simulink model "UDB4_TestBoard"  (Simulink 7.8)
settings: Solver=FixedStepDiscrete  SolverMode=SingleTasking  StartTime=0.0  StopTime=inf  FixedStep=0.001  RelTol=1e-3
libraries: dsPICdrivers x13, simulink x11
settings Model: Creator=Lior  LastModifiedBy=M91449  BufferReuse=off
settings OptimizationCC: BlockReduction=off  InlineParams=on  BufferReuse=off  OptimizeModelRefInitCode=on  LifeSpan=1
settings DebuggingCC: FcnCallInpInsideContextMsg=Use local settings
settings HardwareCC: ProdBitPerInt=16  ProdBitPerPointer=16  ProdEndianess=LittleEndian  ProdWordSize=16  ProdHWDeviceType=16-bit Generic
settings RTWCC: SystemTargetFile=dspic.tlc  MakeCommand=make_CreateMPLAB  TemplateMakefile=dspic_pic30_gcc.tmf  PostCodeGenCommand=dsPIC_Compile()  Description=Embedded Target for Microchip dsPIC (real-time)  ProcessScript=dspic_make_rtw_hook
settings CodeAppCC: IgnoreCustomStorageClasses=off
settings STFCustomTargetCC: IncludeMdlTerminateFcn=off  GeneratePreprocessorConditionals=Use local settings  CombineOutputUpdateFcns=on  SuppressErrorStatus=on  ERTCustomFileBanners=on  SupportContinuousTime=off  SupportNonInlinedSFcns=off  SystemTargetFile=dspic.tlc
settings ERTTargetCC: MultiwordLength=2048  ParMdlRefBuildCompliant=off  CompOptLevelCompliant=off  ConcurrentExecutionCompliant=off  IncludeMdlTerminateFcn=off  SuppressErrorStatus=on  ERTFirstTimeCompliant=off  ModelStepFunctionPrototypeControlCompliant=off  CPPClassGenCompliant=off  ExtModeMexFile=noextcomm  InlinedParameterPlacement=NonHierarchical  ERTSrcFileBannerTemplate=dsPIC_code_template.cgt  ERTHdrFileBannerTemplate=dsPIC_code_template.cgt  ERTDataSrcFileTemplate=dsPIC_code_template.cgt  ERTDataHdrFileTemplate=dsPIC_code_template.cgt  ERTCustomFileTemplate=dsPIC_main.tlc  ConvertIfToSwitch=off  SuppressUnreachableDefaultCases=off
settings CustomProperty: DataType=string  Value=C:\PROGRA~1\MATLAB\R2011B~1\bin\win64\gmake

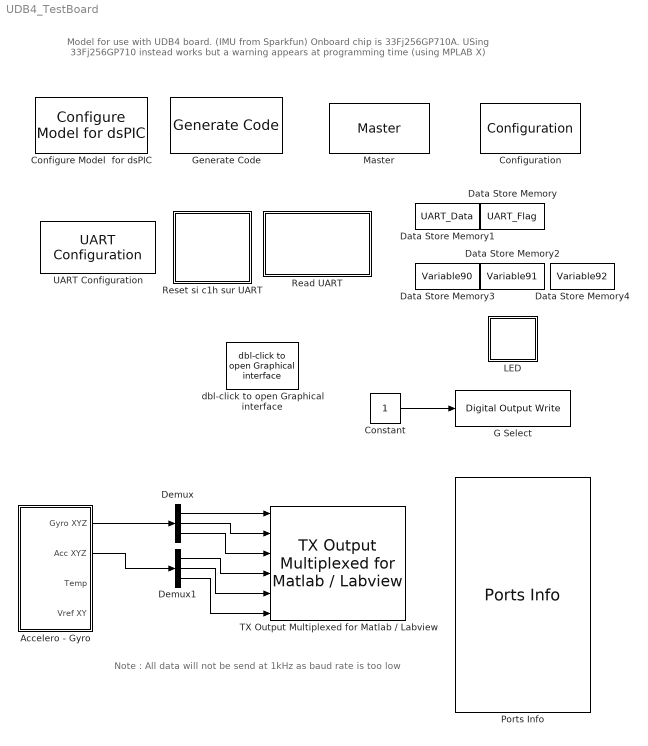
== system UDB4_TestBoard ==
  note: Model for use with UDB4 board. (IMU from Sparkfun)
      | Onboard chip is 33Fj256GP710A.
      | USing 33Fj256GP710 instead works but a warning appears at programming time (using MPLAB X)
  note: Note : All data will not be send at 1kHz as baud rate is too low
  Accelero - Gyro : Subsystem
  Configuration : dsPICdrivers/Configuration  double64=off
  Configure Model  for dsPIC : dsPICdrivers/Simulink Configuration/Configure Model  for dsPIC
  Constant : Constant  OutDataTypeStr=Inherit: Inherit via back propagation
  Data Store Memory : DataStoreMemory  DataStoreName=UART_Flag  ReadBeforeWriteMsg=warning  WriteAfterWriteMsg=warning  WriteAfterReadMsg=warning
  Data Store Memory1 : DataStoreMemory  DataStoreName=UART_Data  ReadBeforeWriteMsg=warning  WriteAfterWriteMsg=warning  WriteAfterReadMsg=warning
  Data Store Memory2 : DataStoreMemory  DataStoreName=Variable91  ReadBeforeWriteMsg=warning  WriteAfterWriteMsg=warning  WriteAfterReadMsg=warning  OutDataTypeStr=uint8
  Data Store Memory3 : DataStoreMemory  DataStoreName=Variable90  ReadBeforeWriteMsg=warning  WriteAfterWriteMsg=warning  WriteAfterReadMsg=warning  OutDataTypeStr=uint8
  Data Store Memory4 : DataStoreMemory  DataStoreName=Variable92  ReadBeforeWriteMsg=warning  WriteAfterWriteMsg=warning  WriteAfterReadMsg=warning  OutDataTypeStr=uint8
  Demux : Demux  Outputs=3
  Demux1 : Demux  Outputs=3
  G Select : dsPICdrivers/Digital I//O/Digital Output Write  Tag=dsPIC_Digital_Output  Priority=5  PORT=A  Pin=6  Simultaneous=on  OrderingInOutPopup=None
  Generate Code : dsPICdrivers/Simulink Configuration/Generate Code
  LED : Subsystem
  Master : dsPICdrivers/Master  Tag=dsPIC_MASTER  Priority=1  TimeStepType=Timer1  picType=33fJ256GP710  fcy=22111111.1111  Quartz_33f=8e6  PLLActive_33f=on  fcyDesired_33f=7.37e6*3  tmr1="[1  22110  0.00050251]"  tmr1Info="Time Step : 0.00099999  ;   Error : 0.00050251%  PR1=22110"  tmr2345="[0  0  0  0  0  0  0  0]"  tmr2345cfg=[-1 -1 -1 -1 -1 -1 -1 -1]  IOautoConf=on  typePort="[ 0   0   0   0   0   0  10   0   0   0   0   0   0   0   0   0   8   8   0   8   8   8   8   8   0   8   8   8   8   0   0   0   0   0   0   0   0   0   0   0   0   0   0   0   0   0   0   0   0   0   0   0   0   0   0   0   0   0   0   0   0   0   0   0   0  10  10  10  10   0   0   0   0   0   0   0   0   0   0   0   0   0   0   0   4   5   0   0   0   0   0   0   0   0   0   0   0   0   0   0   0   0   0   0   0   0   0   0   0   0   0   0 ]"  TRIS="[ 65471  65535  65535  65535  65505  65535  65535 ]"  ADPCFG=507510784  MasterBusyPort=None  MasterOverloadPort=None  FOSC=Quartz (XT - HS)  ClockSwitchMonitor=Clock switching enabled only  TempProtection_33f=TEMP_ON  FPBOR=<empty>  PWRT=disable  MCLR=<empty>  ICD=ICS_PGD1  JTAGEN=JTAGEN_OFF  PowerSave=off  OverrideFcy=off  NewFcy=1e6  PR2345="[65535  65535  65535  65535  65535  65535  65535  65535]"
  Ports Info : dsPICdrivers/Ports Info  Tag=dsPIC_PortInfo
  Read UART : Subsystem  TreatAsAtomicUnit=on
      mask Display: disp('Lecture et\nEnregistrement\nUART')
  Reset si c1h sur UART : Subsystem  TreatAsAtomicUnit=on
      mask Display: disp('Reset\nBootloader')
  TX Output Multiplexed for Matlab / Labview : dsPICdrivers/Serial PORT/TX Output Multiplexed for Matlab // Labview  Tag=dsPIC_TX_Multiplexed  Priority=5  UART=2  CleverSpreadingChk=on  CleverSpreading=1  CHANNEL=[0:5]  CHANNELBLOCKED=[]  CHANNELBLOCKED_BITEWISE=0  Status=OK
  UART Configuration : dsPICdrivers/Serial PORT/UART Configuration  Tag=dsPIC_config_UART  Priority=2  UART=2  proposed_BAUD=Custom  BAUD=115200  ALT_TX_RX=on  InterruptTxWhen=When Transmit Buffer is empty  TXInterruptPri=1  TxBufferSize=32  TXEN=on  InterruptRxWhen=When Receive Buffer is full (contain 4 characters)  RXInterruptPri=2  RxBufferSize=32  DoNotImplementRxInterrupt=off  DoNotImplementTxInterrupt=off  UxBRG=11  Info="UxBRG = 11   ||  Real Baud : 115162   ||  % error : -0.032954  ||  max 11.5162 Bytes / Step"  RealBaud=0  ERROR=-0.032954  BYTES_STEP=11.5162
  dbl-click to open Graphical interface : dsPICdrivers/Serial PORT/dbl-click to open Graphical interface  Nothing=0
  wires:
  Constant/1 -> G Select/1
  Accelero - Gyro/1(Gyro XYZ) -> Demux/1
  Accelero - Gyro/2(Acc XYZ) -> Demux1/1
  Demux/1 -> TX Output Multiplexed for Matlab / Labview/1
  Demux/2 -> TX Output Multiplexed for Matlab / Labview/2
  Demux/3 -> TX Output Multiplexed for Matlab / Labview/3
  Demux1/1 -> TX Output Multiplexed for Matlab / Labview/4
  Demux1/2 -> TX Output Multiplexed for Matlab / Labview/5
  Demux1/3 -> TX Output Multiplexed for Matlab / Labview/6

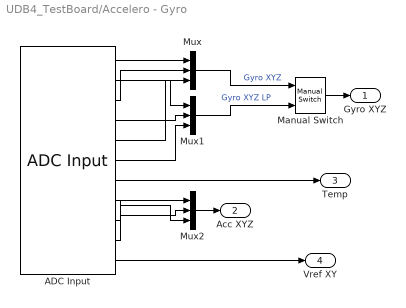
== system UDB4_TestBoard/Accelero - Gyro ==
  ADC Input : dsPICdrivers/Peripheral I//O/ADC Input  Tag=dsPIC_ADC  Priority=5  ADC_TYPE=12 bits  ADC_MODE=Continuous sampling & get last channel value  NbrSampleStep=1  VoltRefpopup="AVdd  -  AVss"  OutFormatBitspopup=0000 dddd dddd dddd : Integer  InterruptPriority=6  ANCHANNELS=[9 10 11 12 0 1 3 4 5 6 7]  MaxName=ANmax = 4095  Rin=1e2  ADCS=29  SAMC=1  Temperature=25  DMAChannel=0  SampleTime=.001  Status="OK  |  Tsmp=6.784e-007 |  T/Channel=1.018e-005 |  Tall=1.119e-004"  SSRC=auto convert
  Manual Switch : simulink/Signal Routing/Manual Switch  sw=1  action=0  varsize=off
  Mux : Mux  Inputs=3
  Mux1 : Mux  Inputs=3
  Mux2 : Mux  Inputs=3
  Gyro XYZ : Outport
  Acc XYZ : Outport  Port=2
  Temp : Outport  Port=3
  Vref XY : Outport  Port=4
  wires:
  ADC Input/1 -> Mux/1
  ADC Input/3 -> Mux/2
  ADC Input/5 -> Mux/3
  ADC Input/2 -> Mux1/1
  ADC Input/4 -> Mux1/2
  ADC Input/6 -> Mux1/3
  ADC Input/10 -> Mux2/1
  ADC Input/9 -> Mux2/2
  ADC Input/8 -> Mux2/3
  Mux/1 -> Manual Switch/1  "Gyro XYZ"
  Mux1/1 -> Manual Switch/2  "Gyro XYZ LP"
  Manual Switch/1 -> Gyro XYZ/1
  ADC Input/7 -> Temp/1
  Mux2/1 -> Acc XYZ/1
  ADC Input/11 -> Vref XY/1

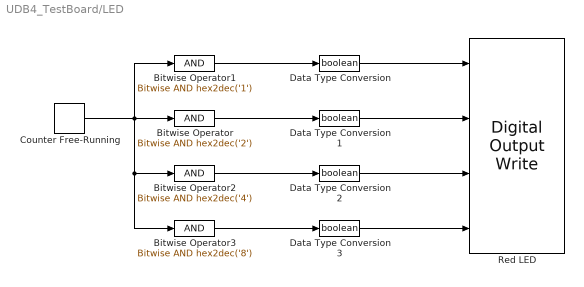
== system UDB4_TestBoard/LED ==
  Bitwise Operator : simulink/Logic and Bit Operations/Bitwise Operator  logicop=AND  UseBitMask=on  BitMask=hex2dec('2')  BitMaskRealWorld=Stored Integer
  Bitwise Operator1 : simulink/Logic and Bit Operations/Bitwise Operator  logicop=AND  UseBitMask=on  BitMask=hex2dec('1')  BitMaskRealWorld=Stored Integer
  Bitwise Operator2 : simulink/Logic and Bit Operations/Bitwise Operator  logicop=AND  UseBitMask=on  BitMask=hex2dec('4')  BitMaskRealWorld=Stored Integer
  Bitwise Operator3 : simulink/Logic and Bit Operations/Bitwise Operator  logicop=AND  UseBitMask=on  BitMask=hex2dec('8')  BitMaskRealWorld=Stored Integer
  Counter Free-Running : simulink/Sources/Counter Free-Running  NumBits=4  tsamp=.1
  Data Type Conversion{,1..3} (4 alike) : DataTypeConversion  OutDataTypeStr=boolean
  Red LED : dsPICdrivers/Digital I//O/Digital Output Write  Tag=dsPIC_Digital_Output  Priority=5  PORT=E  Pin=[1 2 3 4]  Simultaneous=on  OrderingInOutPopup=None
  wires:
  Data Type Conversion/1 -> Red LED/1
  Data Type Conversion1/1 -> Red LED/2
  Data Type Conversion2/1 -> Red LED/3
  Data Type Conversion3/1 -> Red LED/4
  Bitwise Operator1/1 -> Data Type Conversion/1
  Bitwise Operator/1 -> Data Type Conversion1/1
  Bitwise Operator2/1 -> Data Type Conversion2/1
  Bitwise Operator3/1 -> Data Type Conversion3/1
  Counter Free-Running/1 -> Bitwise Operator/1, Bitwise Operator1/1, Bitwise Operator2/1, Bitwise Operator3/1

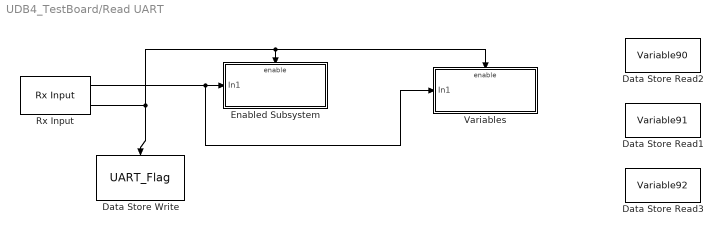
== system UDB4_TestBoard/Read UART ==
  Data Store Read1 : DataStoreRead  DataStoreName=Variable91  SampleTime=.01
  Data Store Read2 : DataStoreRead  DataStoreName=Variable90  SampleTime=.01
  Data Store Read3 : DataStoreRead  DataStoreName=Variable92  SampleTime=.01
  Data Store Write : DataStoreWrite  DataStoreName=UART_Flag
  Enabled Subsystem : Subsystem  TreatAsAtomicUnit=on
  Rx Input : dsPICdrivers/Serial PORT/Rx Input  Tag=dsPIC_RX  Priority=5  UART=2  SampleTime=.01  BlockingFctChk=off  OutputDefault=0  IsPresentFlagChk=on  OrderingInOutPopup=None
  Variables : Subsystem  TreatAsAtomicUnit=on
  wires:
  Rx Input/1 -> Variables/1(In1), Enabled Subsystem/1(In1)
  Rx Input/2 -> Variables/Enable, Enabled Subsystem/Enable, Data Store Write/1

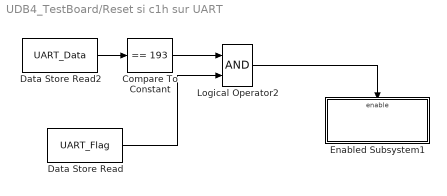
== system UDB4_TestBoard/Reset si c1h sur UART ==
  Compare To Constant : simulink/Logic and Bit Operations/Compare To Constant  relop===  const=193  OutDataTypeStr=boolean  ZeroCross=off
  Data Store Read : DataStoreRead  DataStoreName=UART_Flag
  Data Store Read2 : DataStoreRead  DataStoreName=UART_Data  SampleTime=.01
  Enabled Subsystem1 : Subsystem  TreatAsAtomicUnit=on
  Logical Operator2 : Logic  AllPortsSameDT=off  OutDataTypeStr=boolean
  wires:
  Data Store Read2/1 -> Compare To Constant/1
  Data Store Read/1 -> Logical Operator2/2
  Logical Operator2/1 -> Enabled Subsystem1/Enable
  Compare To Constant/1 -> Logical Operator2/1

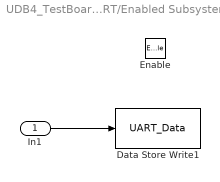
== system UDB4_TestBoard/Read UART/Enabled Subsystem ==
  In1 : Inport
  Enable : EnablePort
  Data Store Write1 : DataStoreWrite  DataStoreName=UART_Data
  wires:
  In1/1 -> Data Store Write1/1

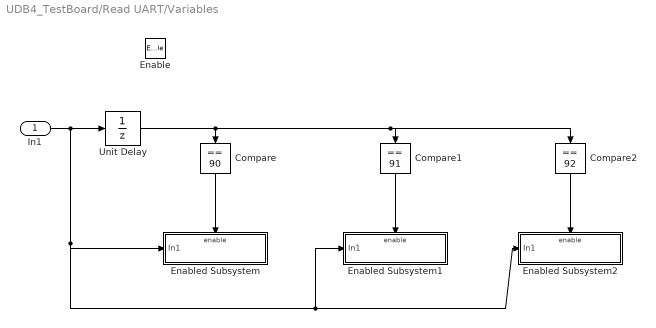
== system UDB4_TestBoard/Read UART/Variables ==
  In1 : Inport
  Enable : EnablePort
  Compare : simulink/Logic and Bit Operations/Compare To Constant  relop===  const=90  OutDataTypeStr=boolean  ZeroCross=off
  Compare1 : simulink/Logic and Bit Operations/Compare To Constant  relop===  const=91  OutDataTypeStr=boolean  ZeroCross=off
  Compare2 : simulink/Logic and Bit Operations/Compare To Constant  relop===  const=92  OutDataTypeStr=boolean  ZeroCross=off
  Enabled Subsystem : Subsystem  TreatAsAtomicUnit=on
  Enabled Subsystem1 : Subsystem  TreatAsAtomicUnit=on
  Enabled Subsystem2 : Subsystem  TreatAsAtomicUnit=on
  Unit Delay : UnitDelay  SampleTime=-1
  wires:
  Compare2/1 -> Enabled Subsystem2/Enable
  Compare1/1 -> Enabled Subsystem1/Enable
  Compare/1 -> Enabled Subsystem/Enable
  Unit Delay/1 -> Compare2/1, Compare1/1, Compare/1
  In1/1 -> Enabled Subsystem2/1(In1), Enabled Subsystem1/1(In1), Enabled Subsystem/1(In1), Unit Delay/1

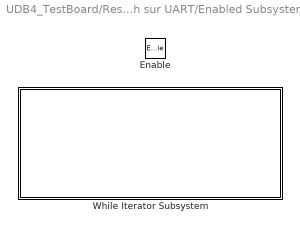
== system UDB4_TestBoard/Reset si c1h sur UART/Enabled Subsystem1 ==
  Enable : EnablePort
  While Iterator Subsystem : Subsystem  TreatAsAtomicUnit=on

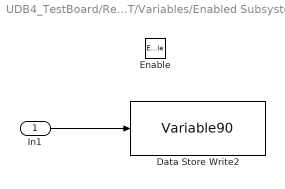
== system UDB4_TestBoard/Read UART/Variables/Enabled Subsystem ==
  In1 : Inport
  Enable : EnablePort
  Data Store Write2 : DataStoreWrite  DataStoreName=Variable90
  wires:
  In1/1 -> Data Store Write2/1

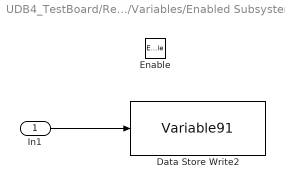
== system UDB4_TestBoard/Read UART/Variables/Enabled Subsystem1 ==
  In1 : Inport
  Enable : EnablePort
  Data Store Write2 : DataStoreWrite  DataStoreName=Variable91
  wires:
  In1/1 -> Data Store Write2/1

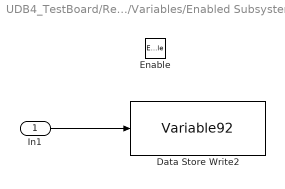
== system UDB4_TestBoard/Read UART/Variables/Enabled Subsystem2 ==
  In1 : Inport
  Enable : EnablePort
  Data Store Write2 : DataStoreWrite  DataStoreName=Variable92
  wires:
  In1/1 -> Data Store Write2/1

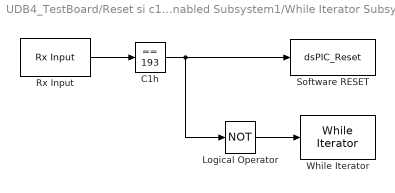
== system UDB4_TestBoard/Reset si c1h sur UART/Enabled Subsystem1/While Iterator Subsystem ==
  C1h : simulink/Logic and Bit Operations/Compare To Constant  relop===  const=193  OutDataTypeStr=boolean  ZeroCross=off
  Logical Operator : Logic  Operator=NOT  AllPortsSameDT=off  OutDataTypeStr=boolean
  Rx Input : dsPICdrivers/Serial PORT/Rx Input  Tag=dsPIC_RX  Priority=5  UART=2  SampleTime=-1  BlockingFctChk=off  OutputDefault=0  IsPresentFlagChk=off  OrderingInOutPopup=None
  Software RESET : S-Function  Tag=dsPIC_Reset  FunctionName=dsPIC_Reset  EnableBusSupport=off
      mask Description: Reset the microcontroller when input is different from 0
      mask Display:
      | fprintf('Reset');
      | port_label('input', 1 ,'~=0');
  While Iterator : WhileIterator  MaxIters=-1  WhileBlockType=do-while  ResetStates=reset
  wires:
  C1h/1 -> Logical Operator/1, Software RESET/1
  Rx Input/1 -> C1h/1
  Logical Operator/1 -> While Iterator/1
